simulink model "Incremental_conductance"  (R2024b)
settings: Solver=VariableStepAuto  StartTime=0.0  StopTime=10.0  MaxStep=1e-4  RelTol=1e-3
libraries: spsPWMGeneratorDCDCLib x1
settings Model: Creator=Abdo  LastModifiedBy=Eng.Abd-Elrhman Saad
settings SolverCC: ZeroCrossAlgorithm=Adaptive  AlgebraicLoopSolver=TrustRegion
settings DataIOCC: ReturnWorkspaceOutputs=off
settings DebuggingCC: MaxConsecutiveZCsMsg=none  UnconnectedInputMsg=warning  UnconnectedOutputMsg=warning  UnconnectedLineMsg=warning  ArithmeticOperatorsInVariantConditions=warning
settings ModelReferenceCC: EnableRefExpFcnMdlSchedulingChecks=on
settings SFSimCC: SimUseLocalCustomCode=off  CustomCodeUndefinedFunction=UseInterfaceOnly
settings RTWCC: RTWUseLocalCustomCode=off  GPUComputeCapability=3.5

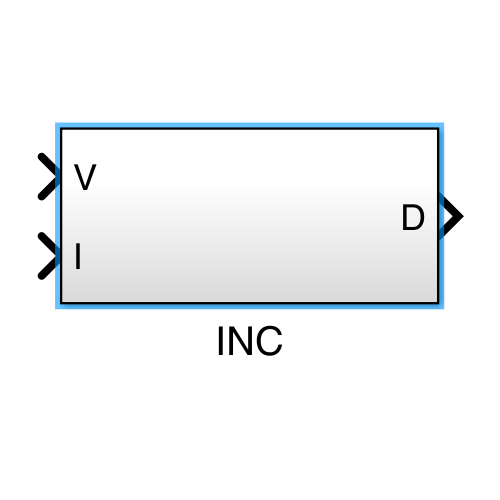
[thumbnail: Simulink's stored preview of the top-level diagram]
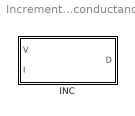
== system Incremental_conductance ==
  INC : Subsystem

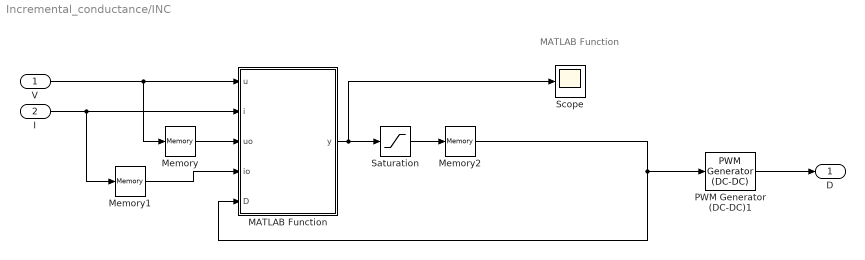
== system Incremental_conductance/INC ==
  note: MATLAB Function
  V : Inport
  I : Inport  Port=2
  MATLAB Function : MATLAB Function  TreatAsAtomicUnit=on
  Memory : Memory  InheritSampleTime=on
  Memory1 : Memory  InheritSampleTime=on
  Memory2 : Memory  InheritSampleTime=on
  PWM Generator (DC-DC)1 : spsPWMGeneratorDCDCLib/PWM Generator (DC-DC)  Fsw=5000  Ts=0
  Saturation : Saturate  UpperLimit=0.95  LowerLimit=0
  Scope : Scope
  D : Outport  VectorParamsAs1DForOutWhenUnconnected=off
  wires:
  Memory/1 -> MATLAB Function/3(uo)
  Saturation/1 -> Memory2/1
  V/1 -> Memory/1, MATLAB Function/1(u)
  Memory1/1 -> MATLAB Function/4(io)
  I/1 -> Memory1/1, MATLAB Function/2(i)
  Memory2/1 -> PWM Generator (DC-DC)1/1, MATLAB Function/5(D)
  MATLAB Function/1(y) -> Scope/1, Saturation/1
  PWM Generator (DC-DC)1/1 -> D/1

== matlab function Incremental_conductance/INC/MATLAB Function ==
  data: u input; y output; i input; uo input; io input; D input
function y = MYMPP(u,i,uo,io,D)
m=0.4;
du=u-uo;
di=i-io;
d=0.00005;
if du==0
    if di==0
    m=D;
    else
        if di>0
            m=D-d;
        else
            m=D+d;
        end
    end
else
    if di/du== -(i/u)
    m=D;
    else
        if di/du> -(i/u)
        m=D-d;
        else
            m=D+d;
        end
    end
end
y = m;
end
